simulink model "mobile_robot_model"  (R2026a)
settings: Solver=ode4  StopTime=60  FixedStep=Ts
values from neighbouring files (symbols this model uses):
  r = 0.045    [init_robot.m]
  Ts = 0.01    [init_robot.m]
  Ts_pos = 1    [init_robot.m]
  x0 = [0; 0; 0]    [init_robot.m]
undefined symbols (not defined in the file or in its folder): sig_pos
libraries: robotmobilelib x1
settings Model: Creator=alemr  LastModifiedBy=alemr

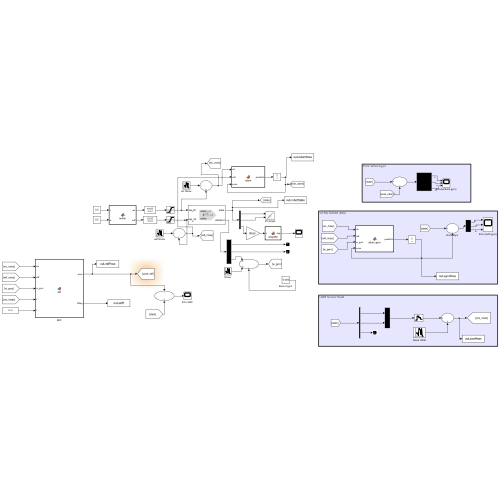
[thumbnail: Simulink's stored preview of the top-level diagram]
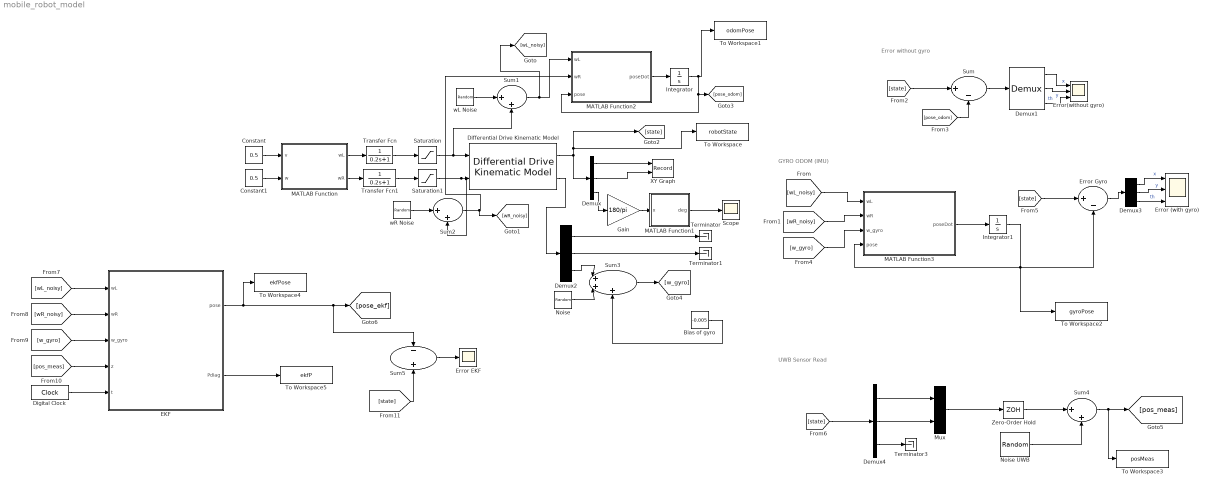
== system mobile_robot_model ==
  note: UWB Sensor Read
  note: GYRO ODOM (IMU)
  note: Error without gyro
  Bias of gyro : Constant  Value=-0.005
  Constant : Constant  Value=0.5
  Constant1 : Constant  Value=0.5
  Demux{,1..4} (5 alike) : Demux  Outputs=3
  Differential Drive Kinematic Model : robotmobilelib/Differential Drive Kinematic Model  VehicleInputs=Wheel Speeds  WheelRadius=r  WheelSpeedRange=[-inf inf]  TrackWidth=L  InitialState=x0  SimulateUsing=Interpreted execution
  Digital Clock : DigitalClock
  EKF : MATLAB Function  TreatAsAtomicUnit=on
  Error (with gyro) : Scope  NumInputPorts=3
      settings: ActiveDisplayYMinimum=-0.41817752039683354  ActiveDisplayYMaximum=0.48492419341552068  DataLoggingVariableName=ScopeData2
  Error EKF : Scope
      settings: ActiveDisplayYMinimum=-0.514118479033611  ActiveDisplayYMaximum=0.43852884784765028  DataLoggingVariableName=ScopeData3
  Error Gyro : Sum  Inputs=|+-
  Error(without gyro) : Scope  NumInputPorts=3
      settings: ActiveDisplayYMinimum=-0.81699802857617132  ActiveDisplayYMaximum=0.7715897168142043
  Gain : Gain  Gain=180/pi
  Integrator : Integrator  InitialCondition=x0
  Integrator1 : Integrator  InitialCondition=x0
  MATLAB Function : MATLAB Function  TreatAsAtomicUnit=on
  MATLAB Function1 : MATLAB Function  TreatAsAtomicUnit=on
  MATLAB Function2 : MATLAB Function  TreatAsAtomicUnit=on
  MATLAB Function3 : MATLAB Function  TreatAsAtomicUnit=on
  Mux : Mux  Inputs=2
  Noise : RandomNumber  Variance=0.0004  Seed=3  SampleTime=Ts
  Noise UWB : RandomNumber  Mean=[0 0]  Variance=[0.01 0.01]  Seed=[4 5]  SampleTime=1
  Saturation : Saturate  UpperLimit=20  LowerLimit=-20
  Saturation1 : Saturate  UpperLimit=20  LowerLimit=-20
  Scope : Scope
      settings: ActiveDisplayYMinimum=-374.93581222580008  ActiveDisplayYMaximum=1012.7958064864923
  Sum : Sum  Inputs=|+-
  Sum1 : Sum  Inputs=|++
  Sum2 : Sum  Inputs=|++
  Sum3 : Sum  Inputs=|+++
  Sum4 : Sum  Inputs=|++
  Sum5 : Sum  Inputs=-+
  Terminator : Terminator
  Terminator1 : Terminator
  Terminator3 : Terminator
  To Workspace : ToWorkspace  VariableName=robotState  SaveFormat=Timeseries  SampleTime=-1
  To Workspace1 : ToWorkspace  VariableName=odomPose  SaveFormat=Timeseries  SampleTime=-1
  To Workspace2 : ToWorkspace  VariableName=gyroPose  SaveFormat=Timeseries  SampleTime=-1
  To Workspace3 : ToWorkspace  VariableName=posMeas  SaveFormat=Timeseries  SampleTime=-1
  To Workspace4 : ToWorkspace  VariableName=ekfPose  SaveFormat=Timeseries  SampleTime=-1
  To Workspace5 : ToWorkspace  VariableName=ekfP  SaveFormat=Timeseries  SampleTime=-1
  Transfer Fcn : TransferFcn  Denominator=[0.2 1]
  Transfer Fcn1 : TransferFcn  Denominator=[0.2 1]
  XY Graph : Record  NumPorts=2.0  FileSettingsInternal="{\"entries\":[{\"content\":{\"excelSettings\":{\"content\":{},\"type\":\"Streamout.ExcelSettings\"},\"parquetSettings\":{\"content\":{},\"type\":\"Streamout.ParquetSettings\"}},\"type\":\"Streamout.FileSettingStorage\",\"uuid\":\"\"}],\"packageUris\":[\"http:\\/\\/schema.mathworks.com\\/mf0\\/streamout_blocks\\/R2020a\"],\"version\":\"1.0\"}"  FrameSettings=[0, 0]  Layout=[1 1]  SignalsInternal="{\"entries\":[{\"content\":{\"signals\":[{\"content\":{\"blockPath\":[],\"dimensions\":[1],\"domain\":\"\",\"lineColor\":\"#a2142f\",\"plots\":[ 1 ],\"port\":1,\"sid\":[\"\"],\"signalID\":1,\"signalName\":\"Demux:1\"},\"type\":\"RecordBlkView.Signal\",\"uuid\":\"\"},{\"content\":{\"blockPath\":[],\"dimensions\":[1],\"domain\":\"\",\"lineColor\":\"#139fff\",\"plots\":[ 1 ],\"port\":2,\"sid\":[\"\"],\"signalID\":2,\"signalName\":\"Demux:2\"},\"type\":\"RecordBlkView.Signal\",\"uuid\":\"\"}]},\"type\":\"RecordBlkView.InputSignals\",\"uuid\":\"\"}],\"packageUris\":[\"http:\\/\\/schema.mathworks.com\\/mf0\\/streamout_blocks\\/R2020a\"],\"version\":\"1.0\"}"  VisualizationBindings="{\"xyplotplugin\":{\"info\":[{\"series\":[{\"bindingParametersList\":[{\"parameter\":\"X-Axis\",\"signalID\":1,\"signalName\":\"Demux:1\"},{\"parameter\":\"Y-Axis\",\"signalID\":2,\"signalName\":\"Demux:2\"}],\"seriesID\":0}],\"subplotID\":1}]}}"  CompatibilityTag=XY
  Zero-Order Hold : ZeroOrderHold
  wL Noise : RandomNumber  Variance=0.25  Seed=1  SampleTime=Ts
  wR Noise : RandomNumber  Variance=0.25  Seed=2  SampleTime=Ts
  wires:
  Demux/1 -> XY Graph/1
  Demux/2 -> XY Graph/2
  Differential Drive Kinematic Model/1 -> To Workspace/1, [state], Demux/1
  MATLAB Function/1(wL) -> Transfer Fcn/1
  MATLAB Function/2(wR) -> Transfer Fcn1/1
  Transfer Fcn/1 -> Saturation/1
  Saturation/1 -> Sum1/2, Differential Drive Kinematic Model/1
  Saturation1/1 -> Sum2/2, Differential Drive Kinematic Model/2
  Transfer Fcn1/1 -> Saturation1/1
  Constant/1 -> MATLAB Function/1(v)
  Constant1/1 -> MATLAB Function/2(w)
  Demux/3 -> Gain/1
  Gain/1 -> MATLAB Function1/1(x)
  MATLAB Function1/1(deg) -> Scope/1
  MATLAB Function2/1(poseDot) -> Integrator/1
  Integrator/1 -> MATLAB Function2/3(pose), [pose_odom], To Workspace1/1
  wL Noise/1 -> Sum1/1
  Sum1/1 -> [wL_noisy], MATLAB Function2/1(wL)
  wR Noise/1 -> Sum2/1
  Sum2/1 -> MATLAB Function2/2(wR), [wR_noisy]
  Differential Drive Kinematic Model/2 -> Demux2/1
  Demux2/1 -> Terminator/1
  Demux2/2 -> Terminator1/1
  Demux2/3 -> Sum3/1
  Noise/1 -> Sum3/2
  Bias of gyro/1 -> Sum3/3
  Sum3/1 -> [w_gyro]
  Demux1/2 -> Error(without gyro)/2  "y"
  [pose_odom] -> Sum/2
  Demux1/1 -> Error(without gyro)/1  "x"
  [state] -> Sum/1
  Demux1/3 -> Error(without gyro)/3  "th"
  Sum/1 -> Demux1/1
  Demux3/2 -> Error (with gyro)/2  "y"
  [wR_noisy] -> MATLAB Function3/2(wR)
  MATLAB Function3/1(poseDot) -> Integrator1/1
  Demux3/3 -> Error (with gyro)/3  "th"
  [state] -> Error Gyro/1
  Integrator1/1 -> To Workspace2/1, MATLAB Function3/4(pose), Error Gyro/2
  [w_gyro] -> MATLAB Function3/3(w_gyro)
  Demux3/1 -> Error (with gyro)/1  "x"
  [wL_noisy] -> MATLAB Function3/1(wL)
  Error Gyro/1 -> Demux3/1
  Zero-Order Hold/1 -> Sum4/1
  Demux4/2 -> Mux/2
  Noise UWB/1 -> Sum4/2
  [state] -> Demux4/1
  Demux4/3 -> Terminator3/1
  Demux4/1 -> Mux/1
  Sum4/1 -> To Workspace3/1, [pos_meas]
  Mux/1 -> Zero-Order Hold/1
  Digital Clock/1 -> EKF/5(t)
  EKF/1(pose) -> To Workspace4/1, Sum5/1, [pose_ekf]
  EKF/2(Pdiag) -> To Workspace5/1
  [wL_noisy] -> EKF/1(wL)
  [wR_noisy] -> EKF/2(wR)
  [w_gyro] -> EKF/3(w_gyro)
  [pos_meas] -> EKF/4(z)
  [state] -> Sum5/2
  Sum5/1 -> Error EKF/1

== matlab function mobile_robot_model/MATLAB Function1 ==
  data: x input; deg output
function deg = wrap360(x)
deg = mod(x, 360);

== matlab function mobile_robot_model/MATLAB Function ==
  data: v input; wL output; w input; wR output
function [wL, wR] = invKin(v, w)
r = 0.045;
L = 0.2194;
wL = (v - w*L/2) / r;
wR = (v + w*L/2) / r;

== matlab function mobile_robot_model/MATLAB Function2 ==
  data: wL input; poseDot output; wR input; pose input
function poseDot = odom(wL, wR, pose)
r = 0.045;
L = 0.2194;
v  = r*(wR + wL)/2;      % forward speed
w  = r*(wR - wL)/L;      % backward speed
th = pose(3);
poseDot = [v*cos(th); v*sin(th); w];

== matlab function mobile_robot_model/MATLAB Function3 ==
  data: wL input; poseDot output; wR input; w_gyro input; pose input
function poseDot = odom_gyro(wL, wR, w_gyro, pose)
r = 0.045;
v  = r*(wR + wL)/2;     
th = pose(3);
poseDot = [v*cos(th); v*sin(th); w_gyro];   % we read omega from gyro sensor

== matlab function mobile_robot_model/EKF ==
  settings: updateMethod=DISCRETE  sampleTime=Ts
  data: wL input; pose output; wR input; w_gyro input; z input; t input; Pdiag output; r parameter; Ts parameter; Ts_pos parameter; sig_pos parameter; x0 parameter
function [pose, Pdiag] = ekf(wL, wR, w_gyro, z, t, r, Ts, Ts_pos, sig_pos, x0)
% process noise
sig_v = 0.02;  % forvard velocity uncertainty
sig_w = 0.03;  % angular velocity uncertainty

persistent xh P
if isempty(xh)
    xh=x0;              % inital guess
    P = diag ([1e-4 1e-4 1e-4 ]);     % certain at the initial
end
%% 1) Prediction ( in every Ts)

v = r*(wR +wL)/2;   % from encoder
w= w_gyro;          % from gyro
th = xh(3);         
xh = xh + [v*cos(th);   v*sin(th);   w]*Ts;


F = [ 1 0 -v*sin(th)*Ts;        % linearization
      0 1 v*cos(th)*Ts;
      0 0 1];

G = [cos(th)*Ts 0;
    sin(th)*Ts 0;
    0 Ts];

Q = G*diag([sig_v^2 sig_w^2])*G';
P = F*P*F' +Q;                        % uncertainty increase

%% 2) Adjusting (only when measure arrives)

if abs(t/Ts_pos - round(t/Ts_pos)) < 1e-6
    H = [1 0 0; 0 1 0];  % sensor only reads x and y
    R = sig_pos^2*eye(2);
    y = z - H*xh;        % measurement - prediction
    S = H*P*H' + R;
    K = P*H'/S;                  % Kalman gain
    xh = xh + K*y;               % adjusting prediciton
    P  = (eye(3) - K*H)*P;       % uncertainty decrease
end

pose = xh;
Pdiag = diag(P);
